simulink subsystem "FromFMtoOmega2"  (R2026a)
settings: Solver=VariableStepAuto
settings Model: Creator=Dell  LastModifiedBy=Carlos Fabian

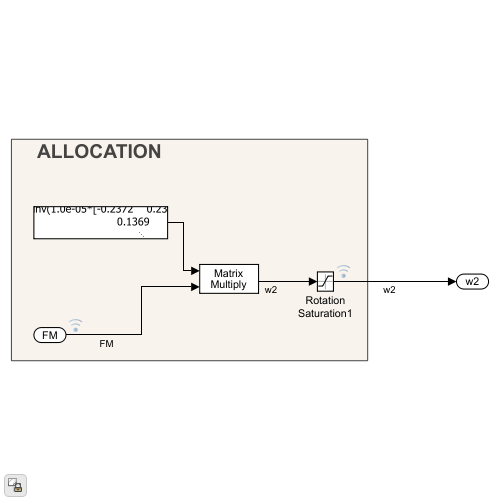
[thumbnail: Simulink's stored preview of the top-level diagram]
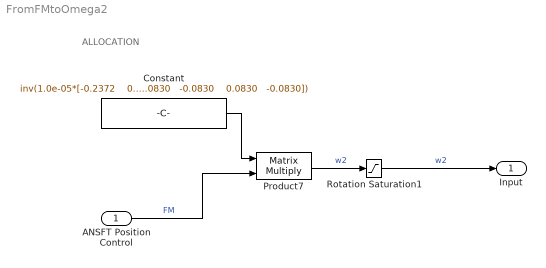
== system FromFMtoOmega2 ==
  note: ALLOCATION
  ANSFT Position Control : Inport
  Constant : Constant  Value=|  SampleTime=0.01
      | inv(1.0e-05*[-0.2372    0.2372    0.0000   -0.2372    0.2372    0.0000;...
      |                      0.1369    0.1369   -0.2739    0.1369    0.1369   -0.2739;...
      |                      0.7525    0.7525    0.7525    0.7525    0.7525    0.7525;...
      |                      0.1694    0.1694    0.0000   -0.1694   -0.1694    0.0000;...
      |                     -0.0978    0.0978    0.1956    0.0978   -0.0978   -0.1956;...
      |                      0.0830   -0.0830    0.0830   -0.0830    0.0830   -0.0830])
  Product7 : Product  Multiplication=Matrix(*)
  Rotation Saturation1 : Saturate  UpperLimit=8.77e+05  LowerLimit=0
  Input : Outport
  wires:
  ANSFT Position Control/1 -> Product7/2  "FM"
  Constant/1 -> Product7/1
  Product7/1 -> Rotation Saturation1/1  "w2"
  Rotation Saturation1/1 -> Input/1  "w2"
